simulink model "top_level"  (R2025b)
settings: Solver=VariableStepAuto  StartTime=0.0  StopTime=10  RelTol=1e-3
libraries: simulink x1
settings Model: Creator=massimoviolante  LastModifiedBy=R
settings ModelReferenceCC: ModelReferenceMinAlgLoopOccurrences=on

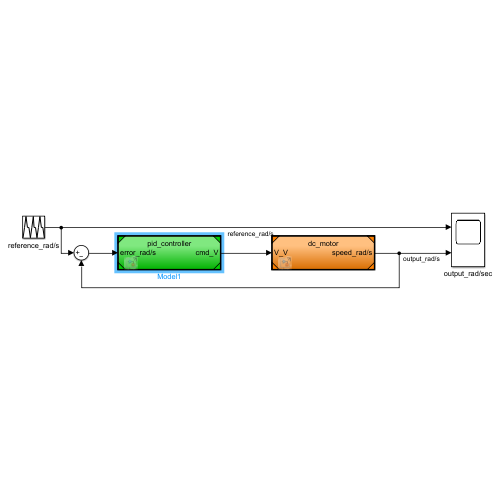
[thumbnail: Simulink's stored preview of the top-level diagram]
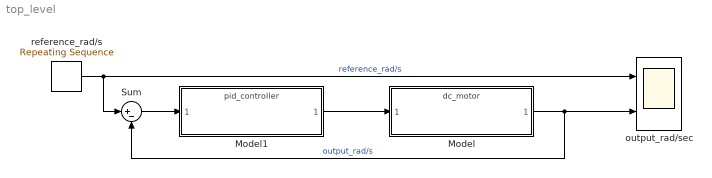
== system top_level ==
  Model : ModelReference  ModelNameDialog=dc_motor.slx  SimulationMode=Normal  ModelReferenceVersion=1.4
  Model1 : ModelReference  ModelNameDialog=pid_controller.slx  SimulationMode=Normal  ModelReferenceVersion=1.3
  Sum : Sum  Inputs=|+-
  output_rad/sec : Scope  NumInputPorts=2
      settings: ActiveDisplayYMinimum=-2.2343155080081711  ActiveDisplayYMaximum=12.156616837744275
  reference_rad/s : simulink/Sources/Repeating Sequence  rep_seq_t=[0 2 4 6 8 10]  rep_seq_y=[0 5 10 5 5 0]
  wires:
  Model/1 -> Sum/2, output_rad/sec/2  "output_rad/s"
  Model1/1 -> Model/1
  Sum/1 -> Model1/1
  reference_rad/s/1 -> Sum/1, output_rad/sec/1  "reference_rad/s"
